simulink model "w5_tlcd_eew"  (R2026a)
settings: Solver=ode4  StopTime=Tend  FixedStep=dt
values from neighbouring files (symbols this model uses):
  C0 = zeros(n+1);  C0(1:n,1:n) = b.C    [w5_sim_run.m]    (also in w5_simulate.m = b.C)
  cA = 0.5 * p.rho * tl.A    [w5_simulate.m]
  g0 = interp1(S.LTA.pga, S.LTA.best_gamma, 0.2)    [w5_main.m]    (also in w5_pump_sens.m; w5_sim_compare.m)
  g1 = interp1(LT.pga, LT.best_gamma, pp)    [w5_main.m]    (also in w5_pump_sens.m = interp1(LT.pga, LT.best_gamma, pga); w5_sim_compare.m = interp1(LT.pga, LT.best_gamma, pga))
  K0 = zeros(n+1);  K0(1:n,1:n) = b.K    [w5_sim_run.m]    (also in w5_simulate.m = b.K)
  kstop = tl.k_stop * kf(i+1)    [w5_simulate.m]
  Lv = [-(b.M + mf*(e*e'))*b.r; -a*mf]    [w5_sim_run.m]
  M = zeros(n+1)    [w5_sim_run.m]    (also in w5_simulate.m = b.M)
  mf = tl.mf    [w5_sim_run.m]    (also in w5_simulate.m)
  tA = tP + 4.5    [w5_fig_records.m]    (also in w5_setting.m = tS - Tlead)
undefined symbols (not defined in the file or in its folder): lxi0, lxi1, rate_g, rate_xi, stroke, w1d
settings Model: Creator=aim88  LastModifiedBy=aim88

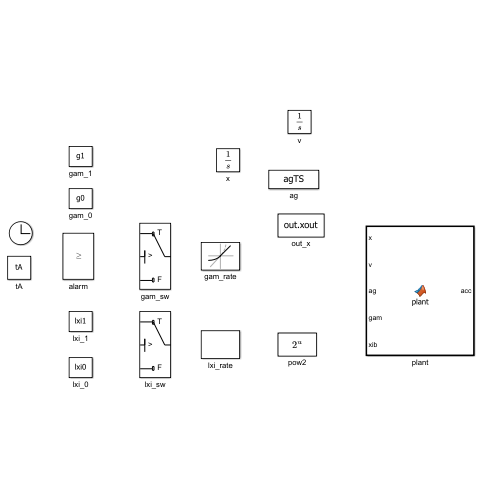
[thumbnail: Simulink's stored preview of the top-level diagram]
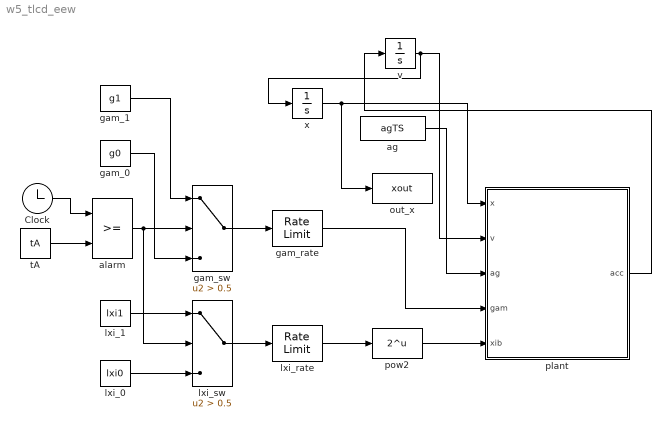
== system w5_tlcd_eew ==
  Clock : Clock
  ag : FromWorkspace  VariableName=agTS
  alarm : RelationalOperator  OutDataTypeStr=boolean  RndMeth=Simplest  InputSameDT=off
  gam_0 : Constant  Value=g0
  gam_1 : Constant  Value=g1
  gam_rate : RateLimiter  RisingSlewLimit=rate_g  FallingSlewLimit=-rate_g  SampleTimeMode=inherited  InitialCondition=g0
  gam_sw : Switch  Criteria=u2 > Threshold  Threshold=0.5  SaturateOnIntegerOverflow=off  InputSameDT=off
  lxi_0 : Constant  Value=lxi0
  lxi_1 : Constant  Value=lxi1
  lxi_rate : RateLimiter  RisingSlewLimit=rate_xi  FallingSlewLimit=-rate_xi  SampleTimeMode=inherited  InitialCondition=lxi0
  lxi_sw : Switch  Criteria=u2 > Threshold  Threshold=0.5  SaturateOnIntegerOverflow=off  InputSameDT=off
  out_x : ToWorkspace  VariableName=xout  SampleTime=-1
  plant : MATLAB Function  TreatAsAtomicUnit=on
  pow2 : Fcn  Expr=2^u
  tA : Constant  Value=tA
  v : Integrator  InitialCondition=zeros(7,1)
  x : Integrator  InitialCondition=zeros(7,1)
  wires:
  gam_1/1 -> gam_sw/1
  alarm/1 -> gam_sw/2, lxi_sw/2
  gam_0/1 -> gam_sw/3
  Clock/1 -> alarm/1
  tA/1 -> alarm/2
  lxi_sw/1 -> lxi_rate/1
  lxi_1/1 -> lxi_sw/1
  gam_sw/1 -> gam_rate/1
  lxi_0/1 -> lxi_sw/3
  x/1 -> plant/1(x), out_x/1
  gam_rate/1 -> plant/4(gam)
  lxi_rate/1 -> pow2/1
  v/1 -> x/1, plant/2(v)
  ag/1 -> plant/3(ag)
  pow2/1 -> plant/5(xib)
  plant/1(acc) -> v/1

== matlab function w5_tlcd_eew/plant ==
  data: x input; acc output; v input; ag input; gam input; xib input; M parameter; K0 parameter; C0 parameter; Lv parameter; mf parameter; cA parameter; w1d parameter; stroke parameter; kstop parameter
function acc = plant(x, v, ag, gam, xib, M, K0, C0, Lv, mf, cA, w1d, stroke, kstop)
% 건물 6층 + TLCD (7자유도) 가속도 — w5_simulate.m 과 같은 식
kf = mf*(gam*w1d)^2;
K = K0;  K(7,7) = kf;
% Δ-DBG: 최상층 변위 증분 부호 = 최상층 속도 부호
if v(6)*v(7) <= 0, xi = 2.0*xib; else, xi = 0.6*xib; end
C = C0;  C(7,7) = cA*xi*abs(v(7));
Fs = zeros(7,1);  ov = abs(x(7)) - stroke;
if ov > 0, Fs(7) = -kstop*kf*ov*sign(x(7)); end
acc = M \ (Lv*ag + Fs - C*v - K*x);
